simulink model "x3DOF_bener"  (R2024b)
settings: Solver=VariableStepAuto  StartTime=0.0  StopTime=250  FixedStep=au  RelTol=1e-10
undefined symbols (not defined in the file): controller, dr2, dr3, du2, du3, dv2, dv3, gamma, Gpi, guidance, IzMinNrd, m, magnitude, Nr, x_8, x_custom, x_elips, x_L, x_ling, x_s, x_sinus, Xu, Xud, y_8, y_custom, y_elips, y_L, y_ling, y_s, y_sinus, Yv, Yvd
libraries: fuzblock x8, simulink x6, mssSimulink x1
(part 2 of 2)

== matlab function x3DOF_bener/Speed Reference Control ==
  settings: updateMethod=DISCRETE
  data: v_actual input; x_current input; x_next input; v_ref output; d_lookahead output; d_next output; v_normal input; t_lookahead input; psi_error output; psi_error input; turning_factor output; cte input
% function [v_ref, d_lookahead, d_next, psi_error, turning_factor] = MATLAB_Function4(v_actual, x_current, x_next, v_normal, t_lookahead, psi_error, cte)
%PROGRAM ASLI
% function [v_ref, d_lookahead, d_next, psi_error, turning_factor] = MATLAB_Function4(v_actual, x_current, x_next, v_normal, t_lookahead, psi_error, cte)
% %% Actual
% function [v_ref, d_lookahead, d_next, psi_error, turning_factor] = MATLAB_Function4(v_actual, x_current, x_next, v_normal, t_lookahead, psi_error, cte)
%     % Parameters
%     v_min = 0.05 * v_normal; % Minimum speed
%     v_stop = 0; % Speed for stopping to correct yaw
%     stop_duration = 10; % Duration to stop (in simulation steps)
%     d_next = norm(x_next - x_current); % Distance to next waypoint
%     psi_error = abs(psi_error); % Absolute yaw error in radians
% 
%     % Dynamic threshold for yaw correction based on psi_error
%     sharp_turn_threshold = deg2rad(15); % Threshold for sharp turns (30 degrees)
%     normal_turn_threshold = deg2rad(15); % Threshold for normal turns (10 degrees)
% 
%     % Automatically set the threshold based on psi_error
%     if psi_error > deg2rad(20) % If yaw error is larger than 20 degrees, switch to 30-degree threshold
%         stop_threshold = sharp_turn_threshold;
%     else
%         stop_threshold = normal_turn_threshold;
%     end
% 
%     % Persistent timer for when v_ref = 0
%     persistent stop_timer;
%     if isempty(stop_timer)
%         stop_timer = 0; % Initialize timer
%     end
% 
%     % Predict lookahead distance
%     d_lookahead = max(0.5, v_actual * t_lookahead); % Minimum lookahead distance
% 
%     % Default v_ref value
%     v_ref = v_normal; % Initial speed set to normal
%     turning_factor = 1;
% 
%     % Large yaw correction: Stop temporarily to correct yaw
%     if psi_error > stop_threshold
%         v_ref = v_stop; % Stop the USV
%         stop_timer = stop_timer + 1; % Count the duration of the stop
%     else
%         stop_timer = 0; % Reset the timer if yaw error is small
%     end
% 
%     % After stopping for a certain duration, return to v_min
%     if stop_timer > stop_duration
%         v_ref = v_min; % Return to minimum speed
%         stop_timer = 0; % Reset the timer
%     end
% 
%     % If yaw error is small, apply turning_factor based on cosine
%     if psi_error <= stop_threshold
%         turning_factor = max(cos(psi_error), 0.1); % Smooth transition
%         if psi_error < deg2rad(5) % Straight path
%             turning_factor = 1;
%         end
% 
%         % Consider lookahead distance to the waypoint
%         if d_lookahead > d_next && cte > abs(0.1)
%             turning_factor = turning_factor * 0.5; % Reduce speed further
%         end
% 
%         % Calculate v_ref with turning_factor
%         v_ref = v_normal * turning_factor;
%     end
% 
%     % Ensure v_ref is within limits
%     v_ref = max(v_min, min(v_normal, v_ref));
% end

% buat tes respon rudder and surge % PROGRAM V_REF = 1.5 M/S
function [v_ref, d_lookahead, d_next, psi_error, turning_factor] = MATLAB_Function4(v_actual, x_current, x_next, v_normal, t_lookahead, psi_error, cte)
    % % Parameters
    % v_min = 0.05 * v_normal; % Minimum speed
    % v_stop = 0; % Speed for stopping to correct yaw

    stop_duration = 10; % Duration to stop (in simulation steps)
    d_next = norm(x_next - x_current); % Distance to next waypoint
    psi_error = abs(psi_error); % Absolute yaw error in radians



    % Dynamic threshold for yaw correction based on psi_error
    sharp_turn_threshold = deg2rad(15); % Threshold for sharp turns (30 degrees)
    normal_turn_threshold = deg2rad(15); % Threshold for normal turns (10 degrees)

    % Automatically set the threshold based on psi_error
    if psi_error > deg2rad(20) % If yaw error is larger than 20 degrees, switch to 30-degree threshold
        stop_threshold = sharp_turn_threshold;
    else
        stop_threshold = normal_turn_threshold;
    end

    % Persistent timer for when v_ref = 0
    persistent stop_timer;
    if isempty(stop_timer)
        stop_timer = 0; % Initialize timer
    end

    % Predict lookahead distance
    d_lookahead = max(0.5, v_actual * t_lookahead); % Minimum lookahead distance

    % Default v_ref value
    v_ref = 1.5; % Initial speed set to normal
    turning_factor = 1;
       % Konstanta
    v_ref = 1.5; % Tetap 1.5 m/s

    % Large yaw correction: Stop temporarily to correct yaw
    if psi_error > stop_threshold
        v_ref = 1.5; % Stop the USV
        stop_timer = stop_timer + 1; % Count the duration of the stop
    else
        stop_timer = 0; % Reset the timer if yaw error is small
    end

    % After stopping for a certain duration, return to v_min
    if stop_timer > stop_duration
        v_ref = 1.5; % Return to minimum speed
        stop_timer = 0; % Reset the timer
    end

    % If yaw error is small, apply turning_factor based on cosine
    if psi_error <= stop_threshold
        turning_factor = max(cos(psi_error), 0.1); % Smooth transition
        if psi_error < deg2rad(5) % Straight path
            turning_factor = 1;
        end

        % Consider lookahead distance to the waypoint
        if d_lookahead > d_next && cte > abs(0.1)
            turning_factor = turning_factor * 0.5; % Reduce speed further
        end

        % Calculate v_ref with turning_factor
        v_ref = 1.5;
    end

    % Ensure v_ref is within limits
    v_ref = 1.5 ;
end

% % function [v_ref, d_lookahead, d_next, psi_error, turning_factor] = MATLAB_Function4(v_actual, x_current, x_next, v_normal, t_lookahead, psi_error, cte)
%     stop_duration = 10; % simulation steps
%     d_next = norm(x_next - x_current); 
%     psi_error = abs(psi_error);
% 
%     sharp_turn_threshold = deg2rad(30);
%     normal_turn_threshold = deg2rad(15);
%     stop_threshold = normal_turn_threshold;
%     if psi_error > deg2rad(20)
%         stop_threshold = sharp_turn_threshold;
%     end
% 
%     persistent stop_timer;
%     if isempty(stop_timer)
%         stop_timer = 0;
%     end
% 
%     d_lookahead = max(0.5, v_actual * t_lookahead); 
%     turning_factor = 1;
% 
%     % Default normal speed
%     v_normal = 1.5;
% 
%     if psi_error > stop_threshold
%         v_ref = 0; % benar-benar berhenti
%         stop_timer = stop_timer + 1;
%     else
%         stop_timer = 0;
%         turning_factor = max(cos(psi_error), 0.1);
%         if psi_error < deg2rad(5)
%             turning_factor = 1;
%         end
% 
%         if d_lookahead > d_next && cte > abs(0.1)
%             turning_factor = turning_factor * 0.5;
%         end
% 
%         v_ref = v_normal * turning_factor;
%     end
% 
%     if stop_timer > stop_duration
%         v_ref = v_normal * 0.5;  % mulai jalan pelan-pelan
%         stop_timer = 0;
%     end
% 
%     % Clamp antara 0 - v_normal
%     v_ref = min(max(v_ref, 0), v_normal);
% end
% 
%

== matlab function x3DOF_bener/Fuzzy PID Surge/MATLAB Function ==
  settings: updateMethod=DISCRETE  sampleTime=0.005
  data: Delta_Kp input; Kp output; Delta_Ki input; Delta_Kd input; Ki output; Kd output
function [Kp,Ki,Kd] = Delta_Gain_surge(Delta_Kp,Delta_Ki,Delta_Kd)
    
    Kp_init = 25; Ki_init = 15; Kd_init = 1;
    
    Kp = Kp_init + Delta_Kp;
    Ki = Ki_init + Delta_Ki;
    Kd = Kd_init + Delta_Kd;
    if Kp < 0
        Kp = 0;
    end
    if Ki < 0
        Ki = 0;
    end
    if Kd < 0
        Kd = 0;
    end
end

== matlab function x3DOF_bener/Fuzzy PID Yaw1/MATLAB Function1 ==
  data: Reference input; Error output; Error_In input
function Error = Checking_Mapping(Reference,Error_In)
    if Reference < 0
        Error = -1*Error_In;
    else
        Error = Error_In;
    end
    Error = wrapToPi(Error);

== matlab function x3DOF_bener/PID Yaw/MATLAB Function2 ==
  data: u input; y output
function y = fcn(u)

y = wrapToPi(u);

== matlab function x3DOF_bener/Fuzzy PID Yaw1/MATLAB Function2 ==
  data: u input; y output
function y = fcn(u)

y = wrapToPi(u);

== matlab function x3DOF_bener/Konversi Sinyal  ==
  data: Throttle input; Tu output; Tv output; Rudder input; Tr output; Vx input
function [Tu,Tv,Tr] = CV(Throttle,Rudder,Vx)
% if Throttle > 40
%     Throttle = 40;
% end
% omega =  6361.9325*(1-exp(-0.47575*Throttle/100));
omega = 880.5976.*(1-exp(-4.2591*(abs(Throttle)/100)));
Tu = 0.0517*omega;
Tv=0;
Tr = 577*(0.02).*1.3.*Vx.^2.*sin(Rudder)*0.8;

== matlab function x3DOF_bener/USV 3 DOF ==
  data: V input; percepatan output size=3; T input; Te input; Yaw input; earth_d output size=3
function [percepatan,earth_d] = usv(V,T,Te,Yaw)

%vektor kecepatan searah sumbu x, y dan yaw
u=V(1);
v=V(2);
r=V(3);
u1 = u;
u2 = v;
u3 = r;
u4 = T(1);
u5 = T(3);

m = 11.8;
%Parameter
Iden = [-29.6348962860344
-40.9001863942293
-17.6979213719311
-44.3102231335245
16.7610566258634
-3.25974680868943
-12.2481062983937
-187.525882383106
242.293583318529
0
0
26.3914216879752
-83.6415289921659
103.872584510861
-0.567968563116999
-31.9512915471382
-0.876330232902557];
%Parameter
Xud = Iden(1);
Yvd = Iden(2);
IzMinNrd = Iden(3);
Xu = Iden(4);
du2 = Iden(5);
du3 = Iden(6);

Yv =  Iden(7);
dv2 = Iden(8);
dv3 =Iden(9);
Yrv = Iden(10);
Yvr = Iden(11);

Nr = Iden(12);
dr2 = Iden(13);
dr3 = Iden(14);
Nrv = Iden(15);
Nvr =Iden(16);
Nvv = Iden(17);

Te1 = Te(1);
Te2 = Te(2);
Te3 = Te(3);

earth_d=[cos(Yaw) -sin(Yaw) 0; sin(Yaw) cos(Yaw) 0; 0 0 1]*V;

u_dot = 1/(m-Xud)*((m-Yvd)*u2*u3 + Xu*u1 + du2*abs(u1)*u1 + du3*(abs(u1)^2)*u1 + u4 + Te1) ;
v_dot = 1/(m-Yvd)*(-(m-Xud)*u1*u3 + Yv*u2 + dv2*abs(u2)*u2 + dv3*(abs(u2)^2)*u2 + Yrv*abs(u3)*u1 + Yvr*abs(u1)*u3 + Te2) ;
r_dot = 1/(IzMinNrd)*(-(m-Yvd)*u2*u1 + (m-Xud)*u1*u2 + Nr*u3 + dr2*abs(u3)*u3 + dr3*(abs(u3)^2)*u3 + Nrv*abs(u3)*u2 + Nvr*abs(u2)*u3 + Nvv*abs(u2)*u2 + u5 + Te3) ;

%Output 
percepatan=[u_dot,v_dot,r_dot]';

== matlab function x3DOF_bener/Backup Tidak Digunakan/3 DOF/MATLAB Function ==
  data: V input; eta_d output; Yaw input
function eta_d = eta(V,Yaw)

eta_d=[cos(Yaw) sin(Yaw) 0; -sin(Yaw) cos(Yaw) 0; 0 0 1]*V;

== matlab function x3DOF_bener/MATLAB Function ==
  settings: updateMethod=DISCRETE
  data: x input; y input
% function realTimePlot(x, y, waypointX, waypointY)
% %#codegen
% coder.extrinsic('figure', 'plot', 'hold', 'grid', 'xlabel', 'ylabel', ...
%     'title', 'set', 'drawnow', 'isempty', 'gcf', 'xlim', 'ylim', 'legend');
% 
% % Persistent variables
% persistent xData yData hPlot fig hWaypoint;
% 
% % Inisialisasi variabel pada iterasi pertama
% if isempty(fig)
%     fig = figure('Name', 'Real-Time Plot', 'NumberTitle', 'off');
%     hold on;
%     grid on;
%     xlabel('X');
%     ylabel('Y');
%     title('Real-Time Plot of X vs Y with Waypoints');
%     xData = [];
%     yData = [];
%     hPlot = plot(NaN, NaN, 'b.-', 'MarkerSize', 10); % Plot lintasan
%     hWaypoint = plot(waypointX, waypointY, 'r--', 'MarkerSize', 1, 'LineWidth', 1); % Plot waypoint
%     legend('USV Path', 'Waypoint');
% end
% 
% % Pastikan dimensi konsisten
% if isrow(x)
%     x = x'; % Pastikan x adalah vektor kolom
% end
% if isrow(y)
%     y = y'; % Pastikan y adalah vektor kolom
% end
% 
% % Tambahkan data baru
% if isempty(xData)
%     xData = x; % Inisialisasi xData jika kosong
%     yData = y; % Inisialisasi yData jika kosong
% else
%     xData = [xData; x]; % Tambahkan data baru sebagai baris baru
%     yData = [yData; y]; % Tambahkan data baru sebagai baris baru
% end
% 
% % Perbarui plot lintasan
% set(hPlot, 'XData', xData, 'YData', yData);
% 
% % Perbarui waypoint (jika berubah)
% set(hWaypoint, 'XData', waypointX, 'YData', waypointY);
% % 
% % % Atur batas sumbu secara otomatis jika perlu
% % xlim([min([xData; waypointX]) - 5, max([xData; waypointX]) + 5]);
% % ylim([min([yData; waypointY]) - 5, max([yData; waypointY]) + 5]);
% 
% % Perbarui jendela plot
% drawnow;
% 
% end

function realTimePlot(x, y)
%#codegen
% Fungsi untuk menampilkan plot real-time dari input x dan y
% Input:
%   x - Nilai input x (titik pada sumbu X)
%   y - Nilai input y (titik pada sumbu Y)

% Deklarasikan fungsi grafik sebagai extrinsic
coder.extrinsic('figure', 'plot', 'hold', 'grid', 'xlabel', 'ylabel', ...
    'title', 'set', 'drawnow', 'isempty', 'gcf', 'xlim', 'ylim');

% Persistent variables
persistent xData yData hPlot fig;

% Inisialisasi variabel pada iterasi pertama
if isempty(fig)
    fig = figure('Name', 'Real-Time Plot', 'NumberTitle', 'off');
    hold on;
    grid on;
    xlabel('X');
    ylabel('Y');
    title('Real-Time Plot of X vs Y');
    xData = [];
    yData = [];
    hPlot = plot(NaN, NaN, 'b.-', 'MarkerSize', 10); % Buat plot awal
end

% Tambahkan data baru
xData = [xData, x];
yData = [yData, y];

% Perbarui plot
set(hPlot, 'XData', xData, 'YData', yData);

% Atur batas sumbu secara otomatis jika perlu
xlim([min(xData) - 1, max(xData) + 1]);
ylim([min(yData) - 1, max(yData) + 1]);

% Perbarui jendela plot
drawnow;

end

== matlab function x3DOF_bener/Backup Tidak Digunakan/Konversi Sinyal 1 ==
  data: Throttle input; Tu output; Tv output; Rudder input; Tr output; Vx input
function [Tu,Tv,Tr] = CV(Throttle,Rudder,Vx)
Kthrust = 0.0201;
Tu= Kthrust*1097.6*(1-exp(-13*abs(Throttle)/100));
Tv=0;
Tr = 18*(6.75*(10^-3)).*1.*Vx.^2.*(Rudder/100);

== matlab function x3DOF_bener/Subsystem/ALOS Guidance ==
  settings: updateMethod=DISCRETE
  data: x input; psi_d output; y input; Delta input; gamma input; R_switch input; xdata input; ydata input; U input; K_f input; h input; x_e output; y_e output; Gpi input
function [psi_d,x_e,y_e]= fcn(x,y,Delta,gamma,R_switch,xdata,ydata,U,K_f,h,Gpi)

% waypoints
wpt.pos.x = xdata;
wpt.pos.y = ydata;

% ALOS guidance law
[psi_d,x_e,y_e] = ALOSpsi(x,y,Delta,gamma,h,R_switch,wpt,U,K_f,Gpi);

end
